simulink model "ex737cruise"  (R2022a)
settings: Solver=VariableStepAuto  StartTime=0.0  StopTime=30.0  RelTol=1e-3
settings Model: Creator=test  LastModifiedBy=noahcurran
settings SolverCC: AlgebraicLoopSolver=TrustRegion
settings DebuggingCC: UnconnectedInputMsg=warning  UnconnectedOutputMsg=warning  UnconnectedLineMsg=warning  SFMachineParentedDataDiag=warning
settings RTWCC: DLArmComputeVersion=19.05

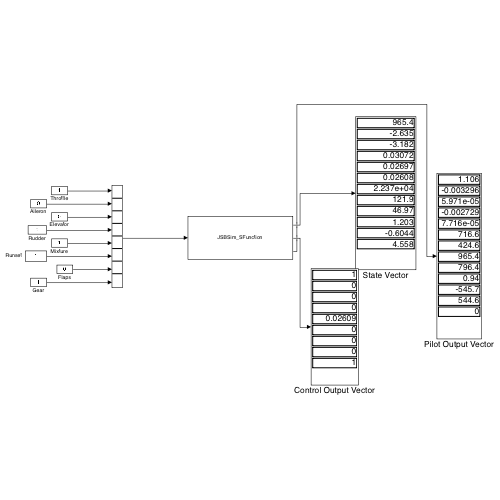
[thumbnail: Simulink's stored preview of the top-level diagram]
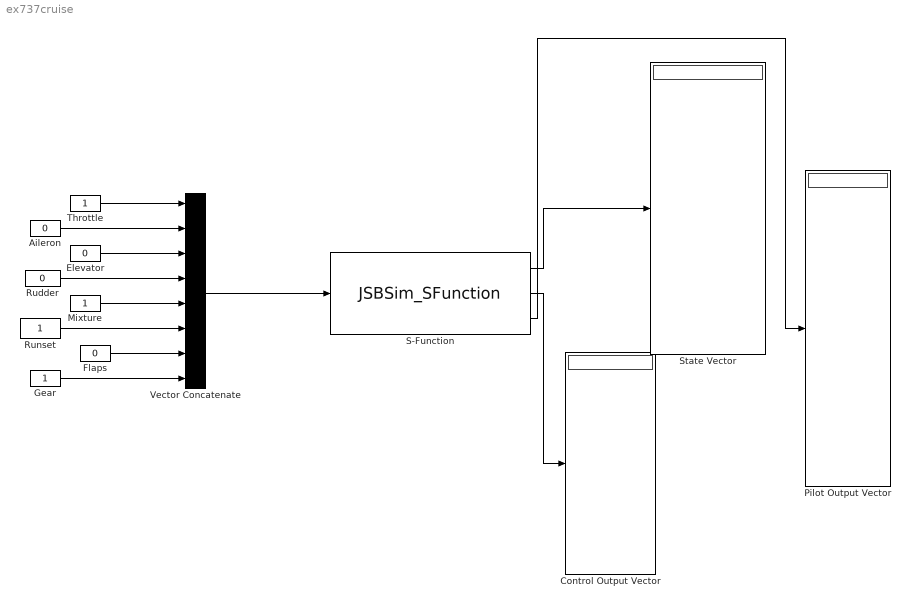
== system ex737cruise ==
  Aileron : Constant  Value=0
  Control Output Vector : Display
  Elevator : Constant  Value=0
  Flaps : Constant  Value=0
  Gear : Constant
  Mixture : Constant
  Pilot Output Vector : Display
  Rudder : Constant  Value=0
  Runset : Constant
  S-Function : S-Function  FunctionName=JSBSim_SFunction  Parameters='737', 0.0083333, 0, 'scripts/737_cruise', 'cruise_init', 'ex737cruise_io'  SFunctionDeploymentMode=off  EnableBusSupport=off
  State Vector : Display
  Throttle : Constant
  Vector Concatenate : Concatenate  NumInputs=8
  wires:
  S-Function/1 -> State Vector/1
  S-Function/3 -> Pilot Output Vector/1
  S-Function/2 -> Control Output Vector/1
  Vector Concatenate/1 -> S-Function/1
  Throttle/1 -> Vector Concatenate/1
  Aileron/1 -> Vector Concatenate/2
  Elevator/1 -> Vector Concatenate/3
  Rudder/1 -> Vector Concatenate/4
  Mixture/1 -> Vector Concatenate/5
  Runset/1 -> Vector Concatenate/6
  Flaps/1 -> Vector Concatenate/7
  Gear/1 -> Vector Concatenate/8
